simulink subsystem "Human_Input_Pre_Processing_sub"  (R2026a)
settings: Solver=VariableStepAuto
undefined symbols (not defined in the file): Rate_Limit_X, Rate_Limit_Y
libraries: simulink x3, sl_discontinuities x2, simulink_need_slupdate x2, Controls_Components_lib x1
settings Model: Creator=ander  LastModifiedBy=ander

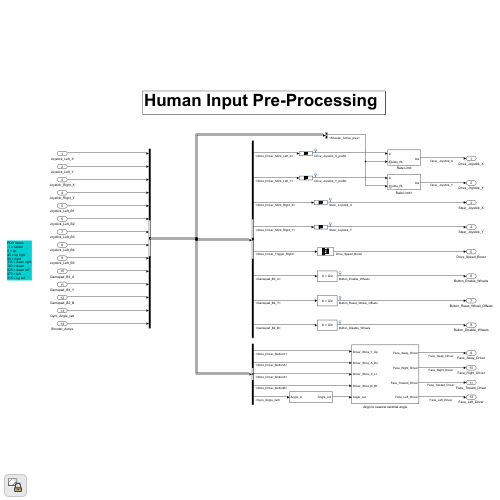
[thumbnail: Simulink's stored preview of the top-level diagram]
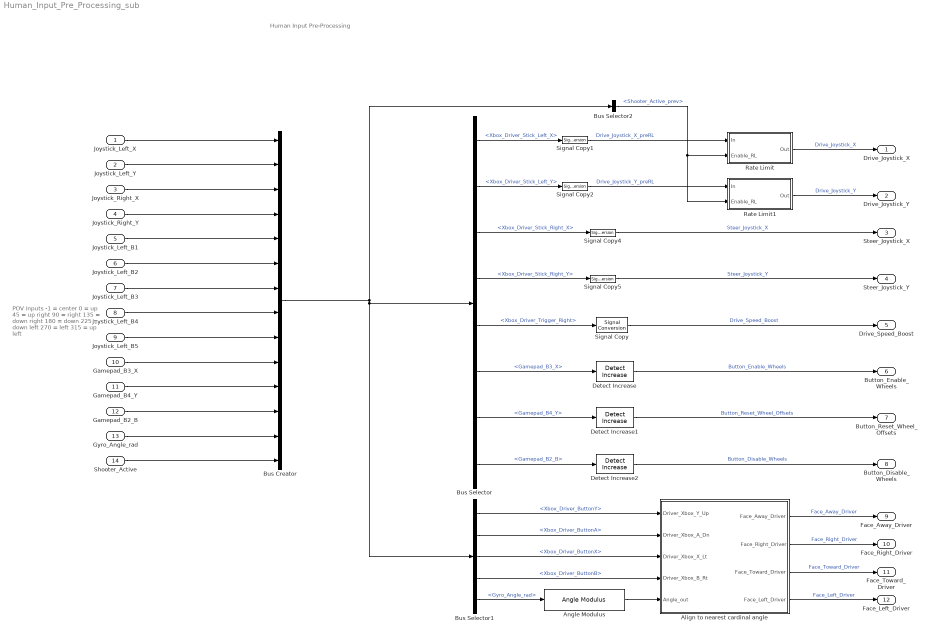
== system Human_Input_Pre_Processing_sub ==
  note: POV inputs
      | -1 = center
      | 0 = up
      | 45 = up right
      | 90 = right
      | 135 = down right
      | 180 = down
      | 225 = down left
      | 270 = left
      | 315 = up left
  note: Human Input Pre-Processing
  Joystick_Left_X : Inport
  Joystick_Left_Y : Inport  Port=2
  Joystick_Right_X : Inport  Port=3
  Joystick_Right_Y : Inport  Port=4
  Joystick_Left_B1 : Inport  Port=5
  Joystick_Left_B2 : Inport  Port=6
  Joystick_Left_B3 : Inport  Port=7
  Joystick_Left_B4 : Inport  Port=8
  Joystick_Left_B5 : Inport  Port=9
  Gamepad_B3_X : Inport  Port=10
  Gamepad_B4_Y : Inport  Port=11
  Gamepad_B2_B : Inport  Port=12
  Gyro_Angle_rad : Inport  Port=13
  Shooter_Active : Inport  Port=14
  Align to nearest cardinal angle : Subsystem
  Angle Modulus : Controls_Components_lib/Angle Modulus  SystemSampleTime=-1  VariantActivationTime=update diagram  EmptyChoice=off  PassThrough=off  PassThroughVariantControl=(default)  EmptyChoiceVariantControl=(default)  AllowFlexibleInterface=on  Latency=0  AutoFrameSizeCalculation=off
  Bus Creator : BusCreator  Inputs=14
  Bus Selector : BusSelector  OutputSignals=Xbox_Driver_Stick_Left_X,Xbox_Driver_Stick_Left_Y,Xbox_Driver_Stick_Right_X,Xbox_Driver_Stick_Right_Y,Xbox_Driver_Trigger_Right,Gamepad_B3_X,Gamepad_B4_Y,Gamepad_B2_B
  Bus Selector1 : BusSelector  OutputSignals=Xbox_Driver_ButtonY,Xbox_Driver_ButtonA,Xbox_Driver_ButtonX,Xbox_Driver_ButtonB,Gyro_Angle_rad
  Bus Selector2 : BusSelector  OutputSignals=Shooter_Active_prev
  Detect Increase : simulink/Logic and Bit Operations/Detect Increase  vinit=0.0  OutDataTypeStr=boolean
  Detect Increase1 : simulink/Logic and Bit Operations/Detect Increase  vinit=0.0  OutDataTypeStr=boolean
  Detect Increase2 : simulink/Logic and Bit Operations/Detect Increase  vinit=0.0  OutDataTypeStr=boolean
  Rate Limit : Subsystem  mask{Rate_Limit=Rate_Limit_X}
  Rate Limit1 : Subsystem  mask{Rate_Limit=Rate_Limit_Y}
  Signal Copy{,1..2,4..5} (5 alike) : SignalConversion  OverrideOpt=off
  Drive_Joystick_X : Outport
  Drive_Joystick_Y : Outport  Port=2
  Steer_Joystick_X : Outport  Port=3
  Steer_Joystick_Y : Outport  Port=4
  Drive_Speed_Boost : Outport  Port=5
  Button_Enable_Wheels : Outport  Port=6
  Button_Reset_Wheel_Offsets : Outport  Port=7
  Button_Disable_Wheels : Outport  Port=8
  Face_Away_Driver : Outport  Port=9
  Face_Right_Driver : Outport  Port=10
  Face_Toward_Driver : Outport  Port=11
  Face_Left_Driver : Outport  Port=12
  wires:
  Bus Creator/1 -> Bus Selector2/1, Bus Selector/1, Bus Selector1/1
  Signal Copy5/1 -> Steer_Joystick_Y/1  "Steer_Joystick_Y"
  Signal Copy4/1 -> Steer_Joystick_X/1  "Steer_Joystick_X"
  Bus Selector/1 -> Signal Copy1/1  "<Xbox_Driver_Stick_Left_X>"
  Bus Selector/2 -> Signal Copy2/1  "<Xbox_Driver_Stick_Left_Y>"
  Bus Selector/3 -> Signal Copy4/1  "<Xbox_Driver_Stick_Right_X>"
  Bus Selector/4 -> Signal Copy5/1  "<Xbox_Driver_Stick_Right_Y>"
  Joystick_Left_X/1 -> Bus Creator/1
  Joystick_Left_Y/1 -> Bus Creator/2
  Bus Selector/6 -> Detect Increase/1  "<Gamepad_B3_X>"
  Bus Selector/7 -> Detect Increase1/1  "<Gamepad_B4_Y>"
  Bus Selector/8 -> Detect Increase2/1  "<Gamepad_B2_B>"
  Detect Increase/1 -> Button_Enable_Wheels/1  "Button_Enable_Wheels"
  Detect Increase1/1 -> Button_Reset_Wheel_Offsets/1  "Button_Reset_Wheel_Offsets"
  Detect Increase2/1 -> Button_Disable_Wheels/1  "Button_Disable_Wheels"
  Signal Copy1/1 -> Rate Limit/1(In)  "Drive_Joystick_X_preRL"
  Signal Copy2/1 -> Rate Limit1/1(In)  "Drive_Joystick_Y_preRL"
  Bus Selector2/1 -> Rate Limit1/2(Enable_RL), Rate Limit/2(Enable_RL)  "<Shooter_Active_prev>"
  Rate Limit/1(Out) -> Drive_Joystick_X/1  "Drive_Joystick_X"
  Rate Limit1/1(Out) -> Drive_Joystick_Y/1  "Drive_Joystick_Y"
  Bus Selector1/5 -> Angle Modulus/1  "<Gyro_Angle_rad>"
  Bus Selector1/1 -> Align to nearest cardinal angle/1(Driver_Xbox_Y_Up)  "<Xbox_Driver_ButtonY>"
  Bus Selector1/3 -> Align to nearest cardinal angle/3(Driver_Xbox_X_Lt)  "<Xbox_Driver_ButtonX>"
  Bus Selector1/4 -> Align to nearest cardinal angle/4(Driver_Xbox_B_Rt)  "<Xbox_Driver_ButtonB>"
  Angle Modulus/1 -> Align to nearest cardinal angle/5(Angle_out)
  Align to nearest cardinal angle/1(Face_Away_Driver) -> Face_Away_Driver/1  "Face_Away_Driver"
  Align to nearest cardinal angle/2(Face_Right_Driver) -> Face_Right_Driver/1  "Face_Right_Driver"
  Align to nearest cardinal angle/3(Face_Toward_Driver) -> Face_Toward_Driver/1  "Face_Toward_Driver"
  Align to nearest cardinal angle/4(Face_Left_Driver) -> Face_Left_Driver/1  "Face_Left_Driver"
  Bus Selector/5 -> Signal Copy/1  "<Xbox_Driver_Trigger_Right>"
  Signal Copy/1 -> Drive_Speed_Boost/1  "Drive_Speed_Boost"
  Bus Selector1/2 -> Align to nearest cardinal angle/2(Driver_Xbox_A_Dn)  "<Xbox_Driver_ButtonA>"
  Gyro_Angle_rad/1 -> Bus Creator/13
  Joystick_Right_Y/1 -> Bus Creator/4
  Gamepad_B2_B/1 -> Bus Creator/12
  Shooter_Active/1 -> Bus Creator/14
  Joystick_Right_X/1 -> Bus Creator/3
  Gamepad_B4_Y/1 -> Bus Creator/11
  Gamepad_B3_X/1 -> Bus Creator/10
  Joystick_Left_B1/1 -> Bus Creator/5
  Joystick_Left_B5/1 -> Bus Creator/9
  Joystick_Left_B4/1 -> Bus Creator/8
  Joystick_Left_B3/1 -> Bus Creator/7
  Joystick_Left_B2/1 -> Bus Creator/6

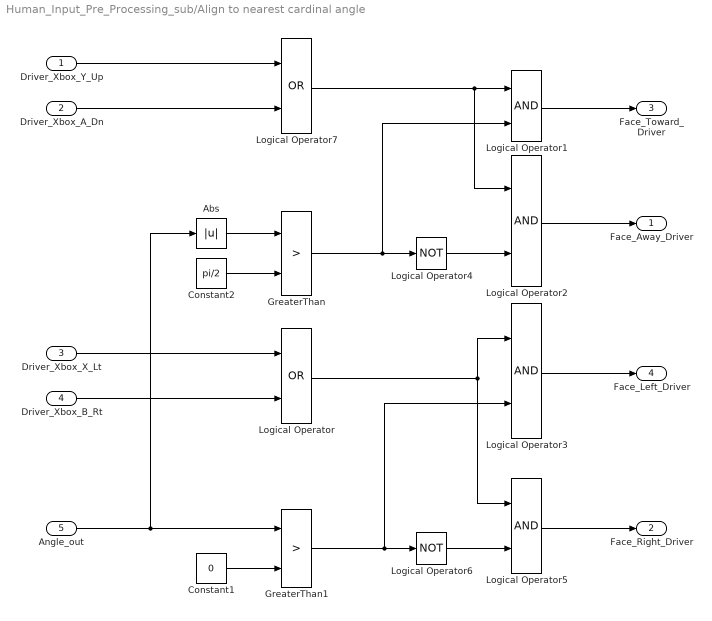
== system Human_Input_Pre_Processing_sub/Align to nearest cardinal angle ==
  Driver_Xbox_Y_Up : Inport
  Driver_Xbox_A_Dn : Inport  Port=2
  Driver_Xbox_X_Lt : Inport  Port=3
  Driver_Xbox_B_Rt : Inport  Port=4
  Angle_out : Inport  Port=5
  Abs : Abs  SaturateOnIntegerOverflow=off
  Constant1 : Constant  Value=0
  Constant2 : Constant  Value=pi/2
  GreaterThan : RelationalOperator  Operator=>  OutDataTypeStr=boolean  RndMeth=Simplest  InputSameDT=off
  GreaterThan1 : RelationalOperator  Operator=>  OutDataTypeStr=boolean  RndMeth=Simplest  InputSameDT=off
  Logical Operator : Logic  Operator=OR  AllPortsSameDT=off  OutDataTypeStr=boolean
  Logical Operator{1..3,5} (4 alike) : Logic  AllPortsSameDT=off  OutDataTypeStr=boolean
  Logical Operator4 : Logic  Operator=NOT  AllPortsSameDT=off  OutDataTypeStr=boolean
  Logical Operator6 : Logic  Operator=NOT  AllPortsSameDT=off  OutDataTypeStr=boolean
  Logical Operator7 : Logic  Operator=OR  AllPortsSameDT=off  OutDataTypeStr=boolean
  Face_Away_Driver : Outport
  Face_Right_Driver : Outport  Port=2
  Face_Toward_Driver : Outport  Port=3
  Face_Left_Driver : Outport  Port=4
  wires:
  Driver_Xbox_A_Dn/1 -> Logical Operator7/2
  Driver_Xbox_Y_Up/1 -> Logical Operator7/1
  Logical Operator5/1 -> Face_Right_Driver/1
  GreaterThan1/1 -> Logical Operator3/2, Logical Operator6/1
  Logical Operator6/1 -> Logical Operator5/2
  Logical Operator4/1 -> Logical Operator2/2
  GreaterThan/1 -> Logical Operator1/2, Logical Operator4/1
  Logical Operator2/1 -> Face_Away_Driver/1
  Logical Operator1/1 -> Face_Toward_Driver/1
  Constant2/1 -> GreaterThan/2
  Abs/1 -> GreaterThan/1
  Logical Operator3/1 -> Face_Left_Driver/1
  Logical Operator/1 -> Logical Operator5/1, Logical Operator3/1
  Constant1/1 -> GreaterThan1/2
  Logical Operator7/1 -> Logical Operator1/1, Logical Operator2/1
  Angle_out/1 -> GreaterThan1/1, Abs/1
  Driver_Xbox_B_Rt/1 -> Logical Operator/2
  Driver_Xbox_X_Lt/1 -> Logical Operator/1

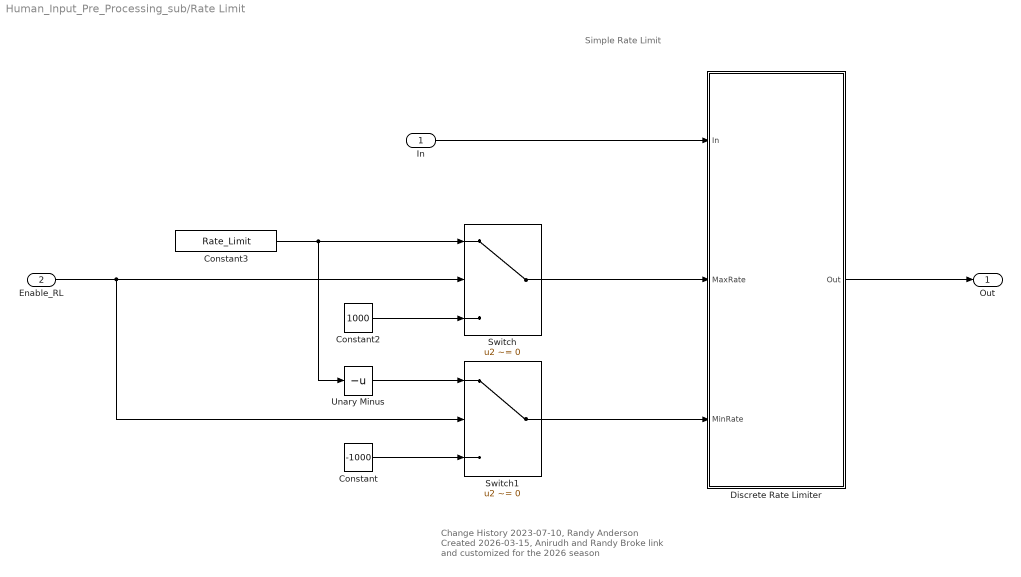
== system Human_Input_Pre_Processing_sub/Rate Limit ==
  note: Change History
      | 2023-07-10, Randy Anderson
      |     Created
      | 2026-03-15, Anirudh and Randy
      |     Broke link and customized for the 2026 season
  note: Simple Rate Limit
  In : Inport
  Enable_RL : Inport  Port=2
  Constant : Constant  Value=-1000
  Constant2 : Constant  Value=1000
  Constant3 : Constant  Value=Rate_Limit
      settings: AttributesFormatString=%<OutDataTypeStr>
  Discrete Rate Limiter : Subsystem
  Switch : Switch  Criteria=u2 ~= 0  SaturateOnIntegerOverflow=off  InputSameDT=off
  Switch1 : Switch  Criteria=u2 ~= 0  SaturateOnIntegerOverflow=off  InputSameDT=off
  Unary Minus : UnaryMinus
  Out : Outport
  wires:
  Unary Minus/1 -> Switch1/1
  Constant2/1 -> Switch/3
  Constant/1 -> Switch1/3
  Switch1/1 -> Discrete Rate Limiter/3(MinRate)
  Switch/1 -> Discrete Rate Limiter/2(MaxRate)
  Enable_RL/1 -> Switch/2, Switch1/2
  Constant3/1 -> Switch/1, Unary Minus/1
  Discrete Rate Limiter/1(Out) -> Out/1
  In/1 -> Discrete Rate Limiter/1(In)

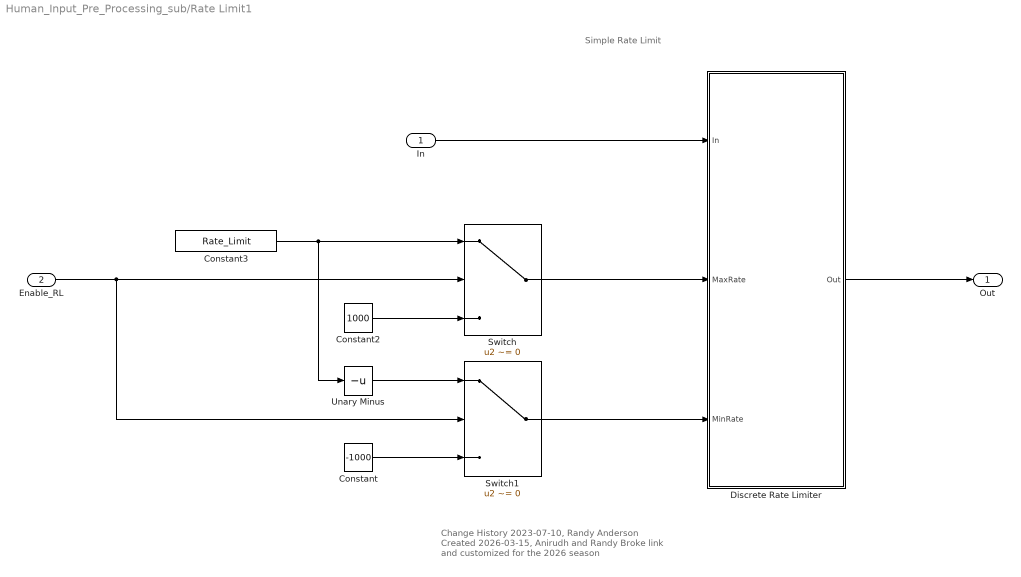
== system Human_Input_Pre_Processing_sub/Rate Limit1 ==
  note: Simple Rate Limit
  note: Change History
      | 2023-07-10, Randy Anderson
      |     Created
      | 2026-03-15, Anirudh and Randy
      |     Broke link and customized for the 2026 season
  In : Inport
  Enable_RL : Inport  Port=2
  Constant : Constant  Value=-1000
  Constant2 : Constant  Value=1000
  Constant3 : Constant  Value=Rate_Limit
      settings: AttributesFormatString=%<OutDataTypeStr>
  Discrete Rate Limiter : Subsystem
  Switch : Switch  Criteria=u2 ~= 0  SaturateOnIntegerOverflow=off  InputSameDT=off
  Switch1 : Switch  Criteria=u2 ~= 0  SaturateOnIntegerOverflow=off  InputSameDT=off
  Unary Minus : UnaryMinus
  Out : Outport
  wires:
  In/1 -> Discrete Rate Limiter/1(In)
  Discrete Rate Limiter/1(Out) -> Out/1
  Constant3/1 -> Unary Minus/1, Switch/1
  Enable_RL/1 -> Switch1/2, Switch/2
  Switch/1 -> Discrete Rate Limiter/2(MaxRate)
  Switch1/1 -> Discrete Rate Limiter/3(MinRate)
  Constant/1 -> Switch1/3
  Constant2/1 -> Switch/3
  Unary Minus/1 -> Switch1/1

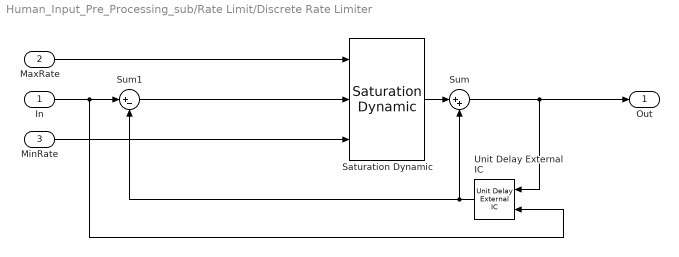
== system Human_Input_Pre_Processing_sub/Rate Limit/Discrete Rate Limiter ==
  In : Inport
  MaxRate : Inport  Port=2
  MinRate : Inport  Port=3
  Saturation Dynamic : sl_discontinuities/Saturation Dynamic  OutMin=[]  OutMax=[]  OutDataTypeStr=Inherit: Same as second input  OutDataType=fixdt(1, 16)  OutScaling=2^-10  DoSatur=off
  Sum : Sum  Inputs=|++  OutDataTypeStr=Inherit: Inherit via back propagation
  Sum1 : Sum  Inputs=|+-  OutDataTypeStr=Inherit: Inherit via back propagation  SaturateOnIntegerOverflow=on
  Unit Delay External IC : simulink_need_slupdate/Unit Delay External IC  tsamp=-1
  Out : Outport
  wires:
  In/1 -> Sum1/1, Unit Delay External IC/2
  Unit Delay External IC/1 -> Sum/2, Sum1/2
  Sum1/1 -> Saturation Dynamic/2
  Saturation Dynamic/1 -> Sum/1
  MaxRate/1 -> Saturation Dynamic/1
  MinRate/1 -> Saturation Dynamic/3
  Sum/1 -> Unit Delay External IC/1, Out/1

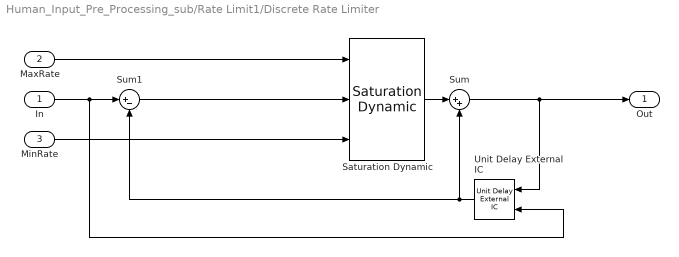
== system Human_Input_Pre_Processing_sub/Rate Limit1/Discrete Rate Limiter ==
  In : Inport
  MaxRate : Inport  Port=2
  MinRate : Inport  Port=3
  Saturation Dynamic : sl_discontinuities/Saturation Dynamic  OutMin=[]  OutMax=[]  OutDataTypeStr=Inherit: Same as second input  OutDataType=fixdt(1, 16)  OutScaling=2^-10  DoSatur=off
  Sum : Sum  Inputs=|++  OutDataTypeStr=Inherit: Inherit via back propagation
  Sum1 : Sum  Inputs=|+-  OutDataTypeStr=Inherit: Inherit via back propagation  SaturateOnIntegerOverflow=on
  Unit Delay External IC : simulink_need_slupdate/Unit Delay External IC  tsamp=-1
  Out : Outport
  wires:
  Sum/1 -> Out/1, Unit Delay External IC/1
  MinRate/1 -> Saturation Dynamic/3
  MaxRate/1 -> Saturation Dynamic/1
  Saturation Dynamic/1 -> Sum/1
  Sum1/1 -> Saturation Dynamic/2
  Unit Delay External IC/1 -> Sum1/2, Sum/2
  In/1 -> Unit Delay External IC/2, Sum1/1
